simulink model "MassSpringDamper_2"  (R2023b)
settings: Solver=VariableStepAuto  StartTime=0.0  StopTime=10.0  RelTol=1e-3
undefined symbols (not defined in the file): X, Y, Z
libraries: sm_lib x8, nesl_utility x7
settings Model: Creator=matte  LastModifiedBy=matte

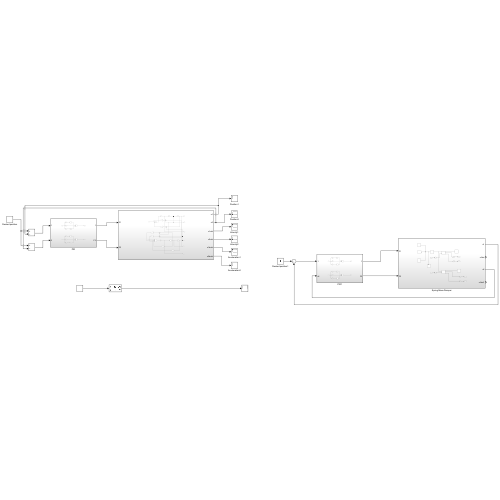
[thumbnail: Simulink's stored preview of the top-level diagram]
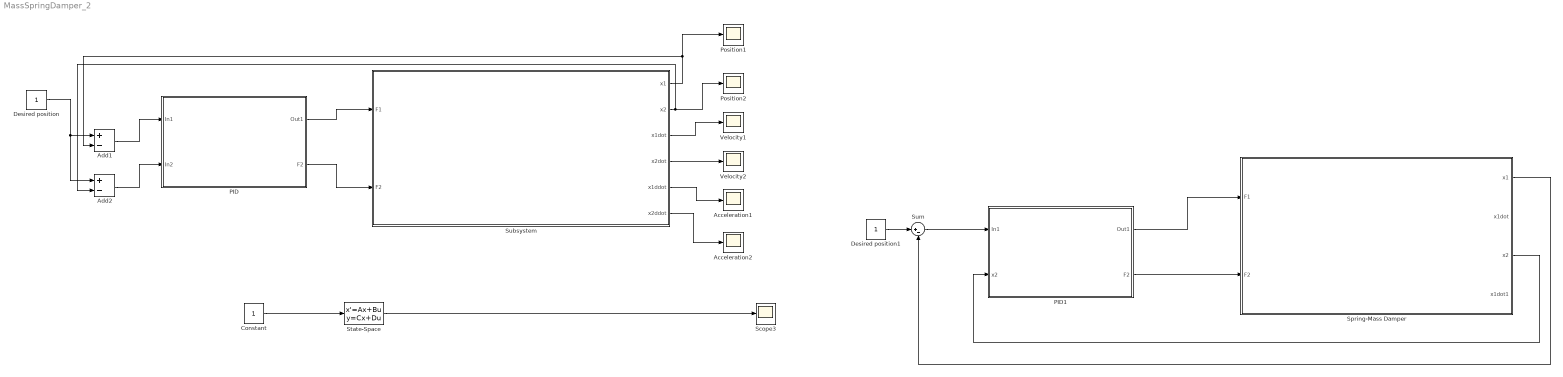
== system MassSpringDamper_2 ==
  Acceleration1 : Scope
  Acceleration2 : Scope
  Add1 : Sum  Inputs=+-
  Add2 : Sum  Inputs=+-
  Constant : Constant
  Desired position : Constant
  Desired position1 : Constant
  PID : Subsystem
  PID1 : Subsystem
  Position1 : Scope
  Position2 : Scope
  Scope3 : Scope
  Spring-Mass Damper : Subsystem
  State-Space : StateSpace  A=[0 0 1 0; 0 0 0 1; -(34)/0.5 20/0.5 -(6.6)/0.5 3.8/0.5; 20 -20 3.8 -3.8]  B=[0 0; 0 0; 1/0.5 0; 0 1]  C=[1 0 0 0; 0 1 0 0]  D=[0 0;0 0]  InitialCondition=0
  Subsystem : Subsystem
  Sum : Sum  Inputs=|+-
  Velocity1 : Scope
  Velocity2 : Scope
  wires:
  Subsystem/4(x2dot) -> Velocity2/1
  Add1/1 -> PID/1(In1)
  PID/1(Out1) -> Subsystem/1(F1)
  Subsystem/6(x2ddot) -> Acceleration2/1
  Constant/1 -> State-Space/1
  Desired position/1 -> Add2/1, Add1/1
  State-Space/1 -> Scope3/1
  Spring-Mass Damper/1(x1) -> Sum/2
  Desired position1/1 -> Sum/1
  Sum/1 -> PID1/1(In1)
  PID/2(F2) -> Subsystem/2(F2)
  Add2/1 -> PID/2(In2)
  Subsystem/1(x1) -> Position1/1, Add1/2
  Subsystem/2(x2) -> Position2/1, Add2/2
  Subsystem/3(x1dot) -> Velocity1/1
  Subsystem/5(x1ddot) -> Acceleration1/1
  PID1/1(Out1) -> Spring-Mass Damper/1(F1)
  PID1/2(F2) -> Spring-Mass Damper/2(F2)
  Spring-Mass Damper/3(x2) -> PID1/2(x2)

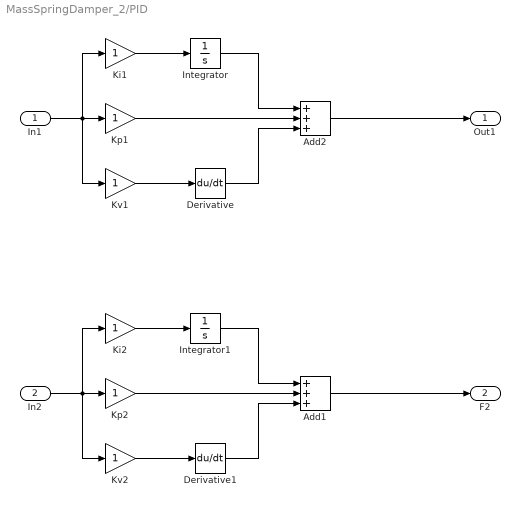
== system MassSpringDamper_2/PID ==
  In1 : Inport
  In2 : Inport  Port=2
  Add1 : Sum  Inputs=+++
  Add2 : Sum  Inputs=+++
  Derivative : Derivative
  Derivative1 : Derivative
  Integrator : Integrator
  Integrator1 : Integrator
  Ki1 : Gain
  Ki2 : Gain
  Kp1 : Gain
  Kp2 : Gain
  Kv1 : Gain
  Kv2 : Gain
  Out1 : Outport
  F2 : Outport  Port=2
  wires:
  Ki1/1 -> Integrator/1
  Kp1/1 -> Add2/2
  Derivative/1 -> Add2/3
  In1/1 -> Kv1/1, Ki1/1, Kp1/1
  Integrator/1 -> Add2/1
  Kv1/1 -> Derivative/1
  Add2/1 -> Out1/1
  In2/1 -> Kv2/1, Ki2/1, Kp2/1
  Integrator1/1 -> Add1/1
  Kv2/1 -> Derivative1/1
  Kp2/1 -> Add1/2
  Derivative1/1 -> Add1/3
  Ki2/1 -> Integrator1/1
  Add1/1 -> F2/1

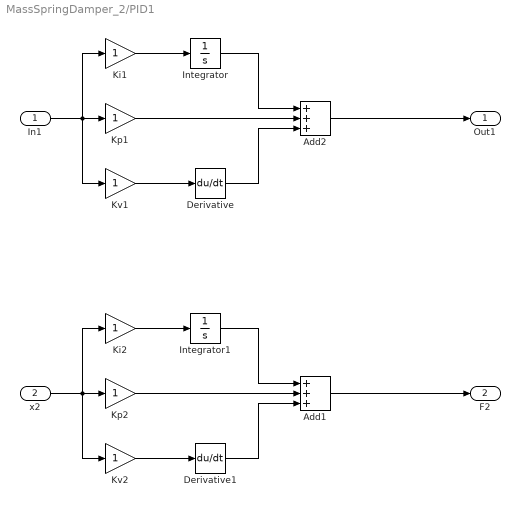
== system MassSpringDamper_2/PID1 ==
  In1 : Inport
  x2 : Inport  Port=2
  Add1 : Sum  Inputs=+++
  Add2 : Sum  Inputs=+++
  Derivative : Derivative
  Derivative1 : Derivative
  Integrator : Integrator
  Integrator1 : Integrator
  Ki1 : Gain
  Ki2 : Gain
  Kp1 : Gain
  Kp2 : Gain
  Kv1 : Gain
  Kv2 : Gain
  Out1 : Outport
  F2 : Outport  Port=2
  wires:
  Ki1/1 -> Integrator/1
  Kp1/1 -> Add2/2
  Derivative/1 -> Add2/3
  In1/1 -> Kv1/1, Ki1/1, Kp1/1
  Integrator/1 -> Add2/1
  Kv1/1 -> Derivative/1
  Add2/1 -> Out1/1
  x2/1 -> Kv2/1, Ki2/1, Kp2/1
  Integrator1/1 -> Add1/1
  Kv2/1 -> Derivative1/1
  Kp2/1 -> Add1/2
  Derivative1/1 -> Add1/3
  Ki2/1 -> Integrator1/1
  Add1/1 -> F2/1

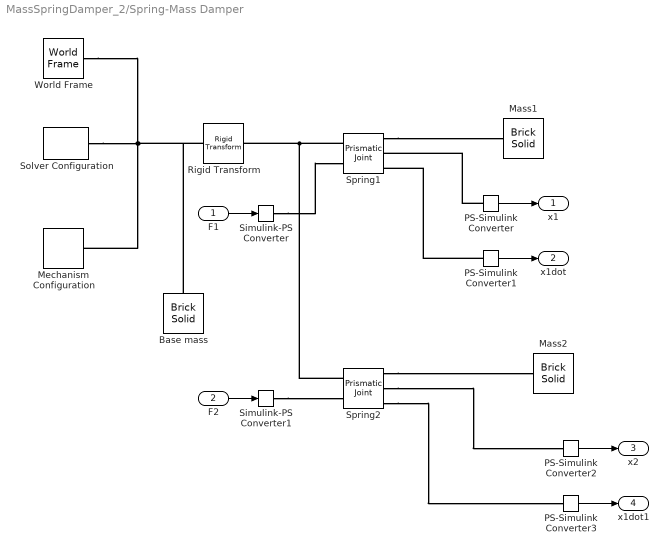
== system MassSpringDamper_2/Spring-Mass Damper ==
  F1 : Inport
  F2 : Inport  Port=2
  Base mass : sm_lib/Body Elements/Brick Solid  GraphicAmbientColor=[0.15 0.15 0.15 1.0]  BasedOnType=Mass  BrickDimensions=[1 1 1]  BrickDimensionsUnits=m  CenterOfMass=[0 0 0]  CenterOfMassUnits=m  GraphicDiffuseColor=[0.5 0.5 0.5]  Density=1000  DensityUnits=kg/m^3  DoExposeReferenceFrame=on  GraphicEmissiveColor=[0.0 0.0 0.0 1.0]  ExportEntireGeometry=off  SerializedFrames=<Frames/>  MarkerShape=Sphere  MarkerSize=10  GraphicType=FromGeometry  InertiaType=CalculateFromGeometry  Mass=1  MassUnits=kg  MomentsOfInertia=[1 1 1]  MomentsOfInertiaUnits=kg*m^2  GraphicOpacity=1.0  ProductsOfInertia=[0 0 0]  ProductsOfInertiaUnits=kg*m^2  GraphicShininess=75  GraphicSpecularColor=[0.5 0.5 0.5 1.0]  GraphicVisPropType=SimpleVisualProperties
  Mass1 : sm_lib/Body Elements/Brick Solid  GraphicAmbientColor=[0.15 0.15 0.15 1.0]  BasedOnType=Mass  BrickDimensions=[1 1 1]  BrickDimensionsUnits=m  CenterOfMass=[0 0 0]  CenterOfMassUnits=m  GraphicDiffuseColor=[0.5 0.5 0.5]  Density=1000  DensityUnits=kg/m^3  DoExposeReferenceFrame=on  GraphicEmissiveColor=[0.0 0.0 0.0 1.0]  ExportEntireGeometry=off  SerializedFrames=<Frames/>  MarkerShape=Sphere  MarkerSize=10  GraphicType=FromGeometry  InertiaType=CalculateFromGeometry  Mass=0.5  MassUnits=kg  MomentsOfInertia=[1 1 1]  MomentsOfInertiaUnits=kg*m^2  GraphicOpacity=1.0  ProductsOfInertia=[0 0 0]  ProductsOfInertiaUnits=kg*m^2  GraphicShininess=75  GraphicSpecularColor=[0.5 0.5 0.5 1.0]  GraphicVisPropType=SimpleVisualProperties
  Mass2 : sm_lib/Body Elements/Brick Solid  GraphicAmbientColor=[0.15 0.15 0.15 1.0]  BasedOnType=Mass  BrickDimensions=[1 1 1]  BrickDimensionsUnits=m  CenterOfMass=[0 0 0]  CenterOfMassUnits=m  GraphicDiffuseColor=[0.5 0.5 0.5]  Density=1000  DensityUnits=kg/m^3  DoExposeReferenceFrame=on  GraphicEmissiveColor=[0.0 0.0 0.0 1.0]  ExportEntireGeometry=off  SerializedFrames=<Frames/>  MarkerShape=Sphere  MarkerSize=10  GraphicType=FromGeometry  InertiaType=CalculateFromGeometry  Mass=1  MassUnits=kg  MomentsOfInertia=[1 1 1]  MomentsOfInertiaUnits=kg*m^2  GraphicOpacity=1.0  ProductsOfInertia=[0 0 0]  ProductsOfInertiaUnits=kg*m^2  GraphicShininess=75  GraphicSpecularColor=[0.5 0.5 0.5 1.0]  GraphicVisPropType=SimpleVisualProperties
  Mechanism Configuration : sm_lib/Utilities/Mechanism Configuration  UniformGravity=Constant  GravityVector=[0 0 -9.80665]  GravityVectorUnits=m/s^2  LinearizationDelta=0.001  JointModeTransitionNonlinearIterations=2
  PS-Simulink Converter{,1..3} (4 alike) : nesl_utility/PS-Simulink Converter  PhysicalDomain=network_engine_domain  SubClassName=ps_output  LeftPortType=input  RightPortType=output  PseudoPeriodic=off  Frequencies=[]  VectorFormat=inherit  Unit=inherit  AffineConversion=off
  Rigid Transform : sm_lib/Frames and Transforms/Rigid Transform  TranslationMethod=StandardAxis  TranslationStandardOffset=15  TranslationStandardOffsetUnits=cm  TranslationStandardAxis=+X  TranslationCartesianOffset=[0 0 0]  TranslationCartesianOffsetUnits=m  TranslationROffset=0  TranslationROffsetUnits=m  TranslationZOffset=0  TranslationZOffsetUnits=m  TranslationThetaOffset=0  TranslationThetaOffsetUnits=deg  RotationMethod=StandardAxis  RotationAngleUnits=deg  RotationStandardAxis=+Y  RotationAngle=90  RotationArbitraryAxis=[0 0 1]  FollAlignAxisA=+X  BaseAlignAxisA=+Y  FollAlignAxisB=+Y  BaseAlignAxisB=+Z  RotationSequenceAxes=FollowerAxes  RotationSequence=XYX  RotationSequenceAngles=[0 0 0]  RotationSequenceAnglesUnits=deg  RotationMatrix=[1 0 0; 0 1 0; 0 0 1]  Quaternion=[1 0 0 0]
  Simulink-PS Converter : nesl_utility/Simulink-PS Converter  PhysicalDomain=network_engine_domain  SubClassName=ps_input  LeftPortType=input  RightPortType=output  PseudoPeriodic=off  Frequencies=[]  NoiseDistribution=none  NoiseParameters=[]  Unit=1  AffineConversion=off  FilteringAndDerivatives=provide  SimscapeFilterOrder=1  InputFilterTimeConstant=0.001  UdotUserProvided=0
  Simulink-PS Converter1 : nesl_utility/Simulink-PS Converter  PhysicalDomain=network_engine_domain  SubClassName=ps_input  LeftPortType=input  RightPortType=output  PseudoPeriodic=off  Frequencies=[]  NoiseDistribution=none  NoiseParameters=[]  Unit=1  AffineConversion=off  FilteringAndDerivatives=provide  SimscapeFilterOrder=1  InputFilterTimeConstant=0.001  UdotUserProvided=0
  Solver Configuration : nesl_utility/Solver Configuration  PhysicalDomain=network_engine_domain  SubClassName=solver  LeftPortType=input  RightPortType=generic  Tones=[]  Harmonics=[]  SimulateNoise=off  Profile=off  UseLocalSampling=off  EnableSwitchedLinearOptims=on  FrequencyDomain=off  UseCCode=off  RelTol=0.001  AbsTol=1e-06  MinStep=1e-09  ToWorkspace=off  RevertToSquareIcSolve=off  NumHomotopyIterations=100  PhasorMode=off  PhasorModeNumHarmonics=1  ConsistencySolver=NEWTON_XTOL_AFTER_FTOL  IndexReductionMethod=DerivativeReplacement  DoDC=off  ResidualTolerance=1e-09  ConsistencyTolSource=GLOBAL  ConsistencyAbsTol=0.001  ConsistencyRelTol=0.001  ConsistencyTolFactor=0.001  UseLocalSolver=off  LocalSolverChoice=NE_BACKWARD_EULER_ADVANCER  ResolveIndetEquations=on  FunctionEvalNumThread=1  LocalSolverSampleTime=0.001  DoFixedCost=off  MaxNonlinIter=3  MaxModeIter=2  ComputeImpulses=off  ImpulseIterations=2  LinearAlgebra=auto  LinearAlgebraNumThread=0  EquationFormulation=NE_TIME_EF  DelaysMemoryBudget=1024  AutomaticFiltering=on  FilteringTimeConstant=0.001  PartitionStorageMethod=AS_NEEDED  PartitionMemoryBudget=1024  PartitionMethod=ROBUST  MultibodyUseLocalSolver=off  MultibodyLocalSolverChoice=ODE1  MultibodyLocalSolverSampleTime=0.001
  Spring1 : sm_lib/Joints/Prismatic Joint  JointMode=Normal  SenseConstraintForce=off  SenseConstraintForceX=off  SenseConstraintForceY=off  SenseConstraintForceZ=off  SenseConstraintTorque=off  SenseConstraintTorqueX=off  SenseConstraintTorqueY=off  SenseConstraintTorqueZ=off  SenseTotalForce=off  SenseTotalForceX=off  SenseTotalForceY=off  SenseTotalForceZ=off  SenseTotalTorque=off  SenseTotalTorqueX=off  SenseTotalTorqueY=off  SenseTotalTorqueZ=off  CompositeWrenchDir=FollowerOnBase  CompositeWrenchFrame=BaseFrame  EquilibriumPosition=10  EquilibriumPositionUnits=cm  SpringStiffness=14  SpringStiffnessUnits=N/m  DampingCoefficient=2.8  DampingCoefficientUnits=N/(m/s)  TorqueActuationMode=InputTorque  MotionActuationMode=ComputedMotion  SensePosition=on  SenseVelocity=on  SenseAcceleration=off  SenseTorqueForce=off  SenseLowerLimitTorqueForce=off  SenseUpperLimitTorqueForce=off  LowerLimitSpecify=off  LowerLimitBound=-1  LowerLimitBoundUnits=m  LowerLimitStiffness=1e6  LowerLimitStiffnessUnits=N/m  LowerLimitDamping=1e3  LowerLimitDampingUnits=N/(m/s)  LowerLimitTransitionRegionWidth=1e-4  LowerLimitTransitionRegionWidthUnits=m  UpperLimitSpecify=off  UpperLimitBound=1  UpperLimitBoundUnits=m  UpperLimitStiffness=1e6  UpperLimitStiffnessUnits=N/m  UpperLimitDamping=1e3  UpperLimitDampingUnits=N/(m/s)  UpperLimitTransitionRegionWidth=1e-4  UpperLimitTransitionRegionWidthUnits=m  PositionTargetSpecify=off  PositionTargetPriority=High  PositionTargetValue=0  PositionTargetValueUnits=m  VelocityTargetSpecify=off  VelocityTargetPriority=High  VelocityTargetValue=0  VelocityTargetValueUnits=m/s
  Spring2 : sm_lib/Joints/Prismatic Joint  JointMode=Normal  SenseConstraintForce=off  SenseConstraintForceX=off  SenseConstraintForceY=off  SenseConstraintForceZ=off  SenseConstraintTorque=off  SenseConstraintTorqueX=off  SenseConstraintTorqueY=off  SenseConstraintTorqueZ=off  SenseTotalForce=off  SenseTotalForceX=off  SenseTotalForceY=off  SenseTotalForceZ=off  SenseTotalTorque=off  SenseTotalTorqueX=off  SenseTotalTorqueY=off  SenseTotalTorqueZ=off  CompositeWrenchDir=FollowerOnBase  CompositeWrenchFrame=BaseFrame  EquilibriumPosition=10  EquilibriumPositionUnits=cm  SpringStiffness=20  SpringStiffnessUnits=N/m  DampingCoefficient=3.8  DampingCoefficientUnits=N/(m/s)  TorqueActuationMode=InputTorque  MotionActuationMode=ComputedMotion  SensePosition=on  SenseVelocity=on  SenseAcceleration=off  SenseTorqueForce=off  SenseLowerLimitTorqueForce=off  SenseUpperLimitTorqueForce=off  LowerLimitSpecify=off  LowerLimitBound=-1  LowerLimitBoundUnits=m  LowerLimitStiffness=1e6  LowerLimitStiffnessUnits=N/m  LowerLimitDamping=1e3  LowerLimitDampingUnits=N/(m/s)  LowerLimitTransitionRegionWidth=1e-4  LowerLimitTransitionRegionWidthUnits=m  UpperLimitSpecify=off  UpperLimitBound=1  UpperLimitBoundUnits=m  UpperLimitStiffness=1e6  UpperLimitStiffnessUnits=N/m  UpperLimitDamping=1e3  UpperLimitDampingUnits=N/(m/s)  UpperLimitTransitionRegionWidth=1e-4  UpperLimitTransitionRegionWidthUnits=m  PositionTargetSpecify=off  PositionTargetPriority=High  PositionTargetValue=0  PositionTargetValueUnits=m  VelocityTargetSpecify=off  VelocityTargetPriority=High  VelocityTargetValue=0  VelocityTargetValueUnits=m/s
  World Frame : sm_lib/Frames and Transforms/World Frame
  x1 : Outport
  x1dot : Outport  Port=2
  x2 : Outport  Port=3
  x1dot1 : Outport  Port=4
  wires:
  PS-Simulink Converter/1 -> x1/1
  F1/1 -> Simulink-PS Converter/1
  PS-Simulink Converter1/1 -> x1dot/1
  F2/1 -> Simulink-PS Converter1/1
  PS-Simulink Converter3/1 -> x1dot1/1
  PS-Simulink Converter2/1 -> x2/1
  connections:
  World Frame/RConn1 -- Solver Configuration/RConn1 -- Mechanism Configuration/RConn1 -- Rigid Transform/LConn1 -- Base mass/RConn1
  Spring1/LConn1 -- Spring2/LConn1 -- Rigid Transform/RConn1
  PS-Simulink Converter/LConn1 -- Spring1/RConn2
  PS-Simulink Converter1/LConn1 -- Spring1/RConn3
  Simulink-PS Converter/RConn1 -- Spring1/LConn2
  Spring1/RConn1 -- Mass1/RConn1
  Simulink-PS Converter1/RConn1 -- Spring2/LConn2
  Spring2/RConn2 -- PS-Simulink Converter2/LConn1
  Spring2/RConn3 -- PS-Simulink Converter3/LConn1
  Spring2/RConn1 -- Mass2/RConn1

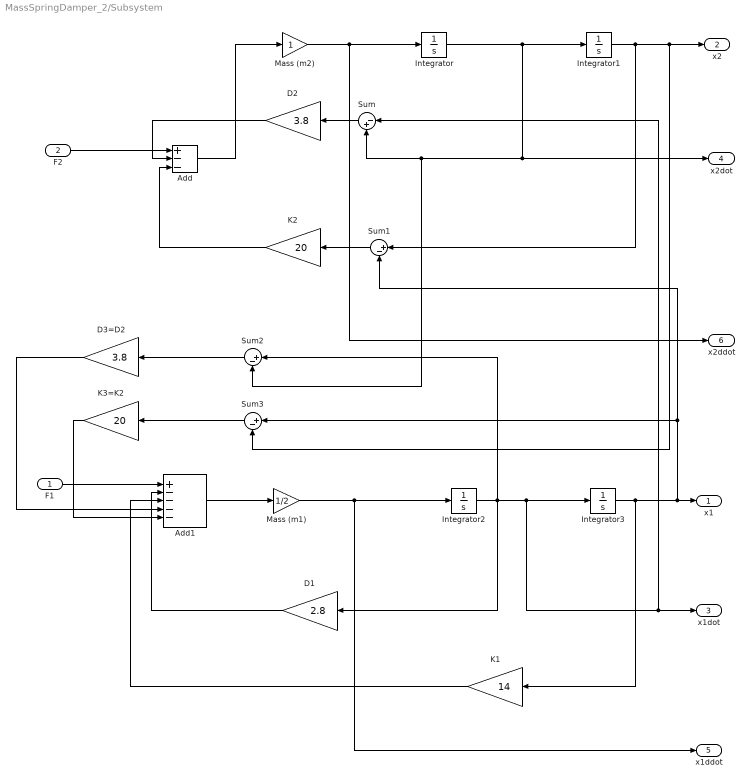
== system MassSpringDamper_2/Subsystem ==
  F1 : Inport
  F2 : Inport  Port=2
  Add : Sum  Inputs=+--
  Add1 : Sum  Inputs=+----
  D1 : Gain  Gain=2.8
  D2 : Gain  Gain=3.8
  D3=D2 : Gain  Gain=3.8
  Integrator{,1..3} (4 alike) : Integrator
  K1 : Gain  Gain=14
  K2 : Gain  Gain=20
  K3=K2 : Gain  Gain=20
  Mass (m1) : Gain  Gain=1/2
  Mass (m2) : Gain
  Sum : Sum  Inputs=|-+
  Sum1 : Sum  Inputs=|+-
  Sum2 : Sum  Inputs=|+-
  Sum3 : Sum  Inputs=|+-
  x1 : Outport
  x2 : Outport  Port=2
  x1dot : Outport  Port=3
  x2dot : Outport  Port=4
  x1ddot : Outport  Port=5
  x2ddot : Outport  Port=6
  wires:
  Integrator1/1 -> Sum1/1, Sum3/2, x2/1
  Integrator/1 -> Integrator1/1, x2dot/1, Sum2/2, Sum/2
  Add/1 -> Mass (m2)/1
  Add1/1 -> Mass (m1)/1
  Mass (m1)/1 -> x1ddot/1, Integrator2/1
  Integrator2/1 -> Sum2/1, D1/1, Sum/1, x1dot/1, Integrator3/1
  F1/1 -> Add1/1
  F2/1 -> Add/1
  D1/1 -> Add1/2
  K1/1 -> Add1/3
  Mass (m2)/1 -> x2ddot/1, Integrator/1
  Sum/1 -> D2/1
  D2/1 -> Add/2
  Integrator3/1 -> K1/1, x1/1, Sum3/1, Sum1/2
  K2/1 -> Add/3
  Sum1/1 -> K2/1
  Sum2/1 -> D3=D2/1
  D3=D2/1 -> Add1/4
  Sum3/1 -> K3=K2/1
  K3=K2/1 -> Add1/5
